simulink model "s_c_nbe_m32k"  (R2018a)
settings: Solver=VariableStepDiscrete  StartTime=0.0  StopTime=1000  RelTol=1e-3
undefined symbols (not defined in the file): fft_stages, n_taps, output_bits, pfb_coeff_gen_calc, xengbits
libraries: xbsIndex_r4 x23714, casper_library_misc x17, xps_library x4, casper_library_scopes x4, xbsReplacements_r4 x4
(part 121 of 171)

== system s_c_nbe_m32k/nb_pfb/pfb_fir_generic1/pfb_fir_taps/sync_delay1 ==
  In : Inport
  en : Inport  Port=2
  Constant : xbsIndex_r4/Constant  const=1  gui_display_data_type=Fixed-point  arith_type=Unsigned  n_bits=BitWidth  bin_pt=0  preci_type=Single  exp_width=8  frac_width=24  explicit_period=on  period=1  equ=P=C  opselect=C  inp2=PCIN>>17  opr=+  inp1=P  carry=CIN  dbl_ovrd=off  block_type=constant
      settings: block_version=9.1.01
  Constant1 : xbsIndex_r4/Constant  const=0  gui_display_data_type=Fixed-point  arith_type=Unsigned  n_bits=BitWidth  bin_pt=0  preci_type=Single  exp_width=8  frac_width=24  explicit_period=on  period=1  equ=P=C  opselect=C  inp2=PCIN>>17  opr=+  inp1=P  carry=CIN  dbl_ovrd=off  block_type=constant
      settings: block_version=9.1.01
  Constant2 : xbsIndex_r4/Constant  const=DelayLen  gui_display_data_type=Fixed-point  arith_type=Unsigned  n_bits=BitWidth  bin_pt=0  preci_type=Single  exp_width=8  frac_width=24  explicit_period=on  period=1  equ=P=C  opselect=C  inp2=PCIN>>17  opr=+  inp1=P  carry=CIN  dbl_ovrd=off  block_type=constant
      settings: block_version=9.1.01
  Constant3 : xbsIndex_r4/Constant  const=UseCounter  gui_display_data_type=Fixed-point  arith_type=Unsigned  n_bits=1  bin_pt=0  preci_type=Single  exp_width=8  frac_width=24  explicit_period=on  period=1  equ=P=C  opselect=C  inp2=PCIN>>17  opr=+  inp1=P  carry=CIN  dbl_ovrd=off  block_type=constant
      settings: block_version=9.1.01
  Counter : xbsIndex_r4/Counter  cnt_type=Free Running  cnt_to=Inf  operation=Down  start_count=0  cnt_by_val=1  arith_type=Unsigned  n_bits=BitWidth  bin_pt=0  load_pin=on  rst=off  en=on  explicit_period=on  period=1  use_behavioral_HDL=off  implementation=Fabric  use_rpm=on  dbl_ovrd=off  block_type=counter
      settings: xl_area=[0, 0, 0, 0, 0, 0, 0]  block_version=9.1.01
  Gateway Out{1..8} (8 alike) : xbsIndex_r4/Gateway Out  inherit_from_input=off  hdl_port=on  rows=1  columns=1  UseAsDAC=off  DACChannel='1'  interface=None  automatic_assignment=on  address_offset=hex2dec('00')  intf_name=''  intf_description=''  timing_constraint=None  locs_specified=off  LOCs={}  io_standard={}  block_type=gatewayout
  Logical : xbsIndex_r4/Logical  logical_function=OR  inputs=2  en=off  latency=0  precision=Full  arith_type=Unsigned  n_bits=8  bin_pt=2  align_bp=on  dbl_ovrd=off  block_type=logical
      settings: xl_area=[0, 0, 0, 0, 0, 0, 0]  block_version=9.1.01
  Logical1 : xbsIndex_r4/Logical  logical_function=AND  inputs=2  en=off  latency=0  precision=Full  arith_type=Unsigned  n_bits=8  bin_pt=2  align_bp=on  dbl_ovrd=off  block_type=logical
      settings: xl_area=[0, 0, 0, 0, 0, 0, 0]  block_version=9.1.01
  Logical2 : xbsIndex_r4/Logical  logical_function=OR  inputs=2  en=off  latency=0  precision=Full  arith_type=Unsigned  n_bits=8  bin_pt=2  align_bp=on  dbl_ovrd=off  block_type=logical
      settings: xl_area=[0, 0, 0, 0, 0, 0, 0]  block_version=9.1.01
  Mux : xbsIndex_r4/Mux  inputs=2  en=off  latency=0  precision=Full  arith_type="Signed  (2's comp)"  n_bits=8  bin_pt=2  quantization=Truncate  overflow=Wrap  dbl_ovrd=off  block_type=mux
      settings: xl_area=[0, 0, 0, 0, 0, 0, 0]  block_version=9.1.01
  Relational : xbsIndex_r4/Relational  mode=a=b  op_type=Bool  en=off  latency=0  dbl_ovrd=off  block_type=relational
      settings: xl_area=[0, 0, 0, 0, 0, 0, 0]  block_version=9.1.01
  Relational1 : xbsIndex_r4/Relational  mode=a!=b  op_type=Bool  en=off  latency=0  dbl_ovrd=off  block_type=relational
      settings: xl_area=[0, 0, 0, 0, 0, 0, 0]  block_version=9.1.01
  To Workspace1 : ToWorkspace  VariableName=tp1  SaveFormat=Timeseries  SampleTime=-1
  To Workspace2 : ToWorkspace  VariableName=tp  SaveFormat=Timeseries  SampleTime=-1
  To Workspace3 : ToWorkspace  VariableName=tp2  SaveFormat=Timeseries  SampleTime=-1
  To Workspace4 : ToWorkspace  VariableName=tp3  SaveFormat=Timeseries  SampleTime=-1
  To Workspace5 : ToWorkspace  VariableName=tp4  SaveFormat=Timeseries  SampleTime=-1
  To Workspace6 : ToWorkspace  VariableName=tp5  SaveFormat=Timeseries  SampleTime=-1
  To Workspace7 : ToWorkspace  VariableName=tp6  SaveFormat=Timeseries  SampleTime=-1
  To Workspace8 : ToWorkspace  VariableName=tp7  SaveFormat=Timeseries  SampleTime=-1
  warn period Logical0 : xbsReplacements_r4/Warning  period=1
  warn period Relational10 : xbsReplacements_r4/Warning  period=1
  Out : Outport
  wires:
  Counter/1 -> Relational1/1, Gateway Out5/1, Relational/2
  Constant1/1 -> Relational1/2
  Constant/1 -> Relational/1
  Constant2/1 -> Counter/2
  In/1 -> Logical2/1, Counter/1, Gateway Out7/1, Mux/2, Logical/1
  Relational1/1 -> Gateway Out3/1, Logical/2
  Relational/1 -> Gateway Out6/1, Mux/3
  Constant3/1 -> Mux/1
  Mux/1 -> Gateway Out8/1, Out/1
  Logical/1 -> Logical1/1, Gateway Out4/1
  en/1 -> Logical1/2, Gateway Out2/1
  Gateway Out2/1 -> To Workspace2/1
  Gateway Out1/1 -> To Workspace1/1
  Gateway Out3/1 -> To Workspace3/1
  Gateway Out4/1 -> To Workspace4/1
  Gateway Out5/1 -> To Workspace5/1
  Gateway Out6/1 -> To Workspace6/1
  Gateway Out7/1 -> To Workspace7/1
  Gateway Out8/1 -> To Workspace8/1
  Logical1/1 -> Logical2/2
  Logical2/1 -> Gateway Out1/1, Counter/3
